simulink model "mcb_ipmsm_fwc_qep_f28379d"  (R2024b)
settings: Solver=FixedStepDiscrete  StartTime=0.0  StopTime=3  RelTol=1e-3  EnableMultiTasking=on
InitFcn:
  | mcb_ipmsm_fwc_qep_f28379d_data;
model workspace (MAT data in the model file):
  encoderResolution = 2000
  hallOffset = '0.5'
  indexOffset = 850
  polePairs = '4'
values from neighbouring files (symbols this model uses):
  dataType = 'single'    [mcb_e11_nonlin_fwc_data.m]    (also in mcb_e11_nonlin_setup.m; mcb_e11_params.m; mcb_ipmsm_fwc_qep_f28379d_data.m)
  inverter =     [e11_pmsmlut_full.mat]    (also in mcb_e11_nonlin_fwc_data.m = mcb_SetInverterParameters('BoostXL-DRV8305'); mcb_e11_nonlin_setup.m = S.inverter; mcb_ipmsm_fwc_qep_f28379d_data.m = mcb_SetInverterParameters('BoostXL-DRV8305'))
  lambda_pm = 0.0758825560532    [e11_pmsm_lut_data.mat]
  maxMotorCurrent = pmsm.I_rated    [mcb_e11_nonlin_fwc_data.m]    (also in mcb_e11_nonlin_setup.m; mcb_ipmsm_fwc_qep_f28379d_data.m)
  PI_params = mcb_SetControllerParameters(pmsm, inverter, PU_System, T_pwm, Ts, Ts_speed, Delays)    [mcb_e11_nonlin_fwc_data.m]    (also in mcb_e11_nonlin_setup.m; mcb_ipmsm_fwc_qep_f28379d_data.m = mcb_SetControllerParameters(pmsm,inverter,PU_System,T_pwm,Ts)
  pmsm = struct('I_rated', 433)    [e11_build_pmsmlut.m]    (also in e11_pmsmlut_full.mat = ; mcb_e11_nonlin_fwc_data.m = mcbPMSMUpdateLdLqFluxPM(pmsm, PMSMLUT, round(tmpmat(1,1)), r; mcb_e11_nonlin_setup.m = S.pmsm; mcb_ipmsm_fwc_qep_f28379d_data.m = mcb_SetPMSMMotorParameters('e11'))
  PU_System = mcb_SetPUSystem(pmsm, inverter)    [mcb_e11_nonlin_fwc_data.m]    (also in mcb_e11_nonlin_setup.m = struct(); mcb_ipmsm_fwc_qep_f28379d_data.m = mcb_SetPUSystem(pmsm,inverter))
  target = mcb_SetProcessorDetails('F28379D',PWM_frequency)    [mcb_ipmsm_fwc_qep_f28379d_data.m]
  Ts = T_pwm    (= 5e-05)    [mcb_e11_nonlin_fwc_data.m]    (also in mcb_e11_nonlin_setup.m; mcb_e11_params.m = ELEC.T_pwm; mcb_ipmsm_fwc_qep_f28379d_data.m)
  Ts_motor = T_pwm/2    (= 2.5e-05)    [mcb_e11_nonlin_fwc_data.m]    (also in mcb_e11_nonlin_setup.m; mcb_e11_params.m = ELEC.T_pwm/2; mcb_ipmsm_fwc_qep_f28379d_data.m)
  Ts_simulink = T_pwm/2    (= 2.5e-05)    [mcb_e11_nonlin_fwc_data.m]    (also in mcb_e11_nonlin_setup.m; mcb_e11_params.m = ELEC.T_pwm/2; mcb_ipmsm_fwc_qep_f28379d_data.m)
  Ts_speed = 30*Ts    (= 0.0015)    [mcb_e11_nonlin_fwc_data.m]    (also in mcb_e11_nonlin_setup.m; mcb_e11_params.m = 30*Ts; mcb_ipmsm_fwc_qep_f28379d_data.m)
undefined symbols (not defined in the file or in its folder): Down, GPTRIP1SEL, GPTRIP2SEL, TZ1, TZ2, Up
libraries: mcbcontrolslib x13, simulink x11, c280xlib x8, c2802xlib x7, slpidlib x4, mcbpositiondecoderlib x3, c2837xDlib x3, mcbpmsmnonlinearlib x2, svdschedulerlib x2, svdutilitieslib x1, mcbplantlib x1, autolibpmsminterior x1
(part 1 of 3)
settings Model: ExtModeTrigDuration=8  Creator=The MathWorks, Inc.  LastModifiedBy=The MathWorks, Inc.
settings SolverCC: AlgebraicLoopSolver=TrustRegion  MaxZcPerStep=1
settings DataIOCC: LimitDataPoints=on  SaveFormat=Array  SaveOutput=off  SaveTime=off  ReturnWorkspaceOutputs=off
settings OptimizationCC: DefaultUnderspecifiedDataType=single  OptimizeBlockIOStorage=off  BufferReuse=off  GlobalBufferReuse=off  ExpressionFolding=off  ExpressionDepthLimit=2147483647  LocalBlockOutputs=off  InitFltsAndDblsToZero=on  NoFixptDivByZeroProtection=on  EfficientFloat2IntCast=on  EfficientMapNaN2IntZero=off  LifeSpan=Inf  MaxStackSize=1024  OptimizeDataStoreBuffers=off  BusAssignmentInplaceUpdate=off  DenormalBehavior=FlushToZero  EfficientTunableParamExpr=on
settings DebuggingCC: ReadBeforeWriteMsg=DisableAll  WriteAfterWriteMsg=DisableAll  WriteAfterReadMsg=DisableAll  CheckSSInitialOutputMsg=off  SignalResolutionControl=TryResolveAllWithWarning  SolverPrmCheckMsg=warning  InheritedTsInSrcMsg=none  MultiTaskDSMMsg=none  MultiTaskCondExecSysMsg=none  TasksWithSamePriorityMsg=none  SigSpecEnsureSampleTimeMsg=none  IntegerOverflowMsg=none  ParameterPrecisionLossMsg=none  FcnCallInpInsideContextMsg=warning  UnconnectedInputMsg=warning  UnconnectedOutputMsg=warning  UnconnectedLineMsg=warning  AllowSymbolicDim=off  StateNameClashWarn=warning  SFUnexpectedBacktrackingDiag=warning  SFNoUnconditionalDefaultTransitionDiag=warning  SFExecutionAtInitializationDiag=none  IntegerSaturationMsg=none  ArithmeticOperatorsInVariantConditions=warning
settings HardwareCC: ProdBitPerChar=16  ProdBitPerInt=16  ProdBitPerPointer=32  ProdBitPerSizeT=32  ProdBitPerPtrDiffT=32  ProdLargestAtomicInteger=Integer  ProdLargestAtomicFloat=None  ProdWordSize=16  ProdLongLongMode=on  ProdHWDeviceType=Texas Instruments->C2000  TargetBitPerChar=16  TargetBitPerInt=16  TargetBitPerPointer=16  TargetLargestAtomicInteger=Integer  TargetIntDivRoundTo=Zero  TargetEndianess=LittleEndian  TargetWordSize=16  TargetHWDeviceType=TI C2000
settings ModelReferenceCC: EnableRefExpFcnMdlSchedulingChecks=on  PropagateSignalLabelsOutOfModel=off
settings SFSimCC: SimUseLocalCustomCode=off  MATLABDynamicMemAlloc=off  CustomCodeUndefinedFunction=UseInterfaceOnly
settings RTWCC: Description=Embedded Coder  SystemTargetFile=ert.tlc  HardwareBoard=TI Delfino F28379D LaunchPad  TemplateMakefile=ert_default_tmf  GenerateReport=on  RTWUseLocalCustomCode=off  Toolchain=Texas Instruments Code Composer Studio (C2000)  IncludeHyperlinkInReport=on  LaunchReport=on  GenerateTraceInfo=on  GenerateTraceReport=on  GenerateTraceReportSl=on  GenerateTraceReportSf=on  GenerateTraceReportEml=on  GPUComputeCapability=3.5  DLArmComputeVersion=19.05
settings CodeAppCC: IgnoreCustomStorageClasses=off  CustomSymbolStrType=$N$R$M  StateflowObjectComments=on  InternalIdentifier=Classic
settings ERTTargetCC: CodeReplacementLibrary=TI C28x  MultiwordLength=2048  ExtModeStaticAllocSize=10000  InlinedParameterPlacement=Hierarchical  ConvertIfToSwitch=off  SuppressUnreachableDefaultCases=off  MemSecPackage=tic2000demospkg
settings ConfigComp: CovMetricSettings=dw  CovSaveCumulativeToWorkspaceVar=on  CovSaveSingleToWorkspaceVar=on  CovExternalEMLEnable=off  CovSFcnEnable=off

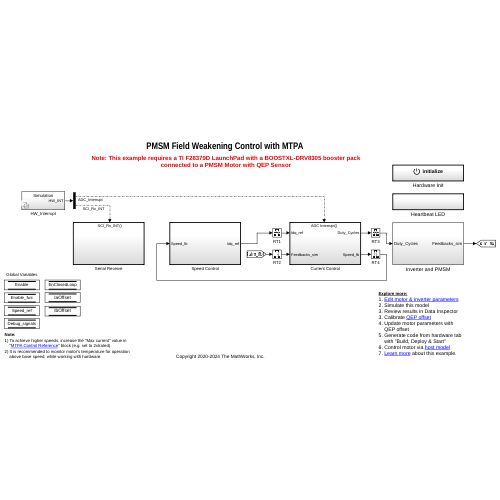
[thumbnail: Simulink's stored preview of the top-level diagram]
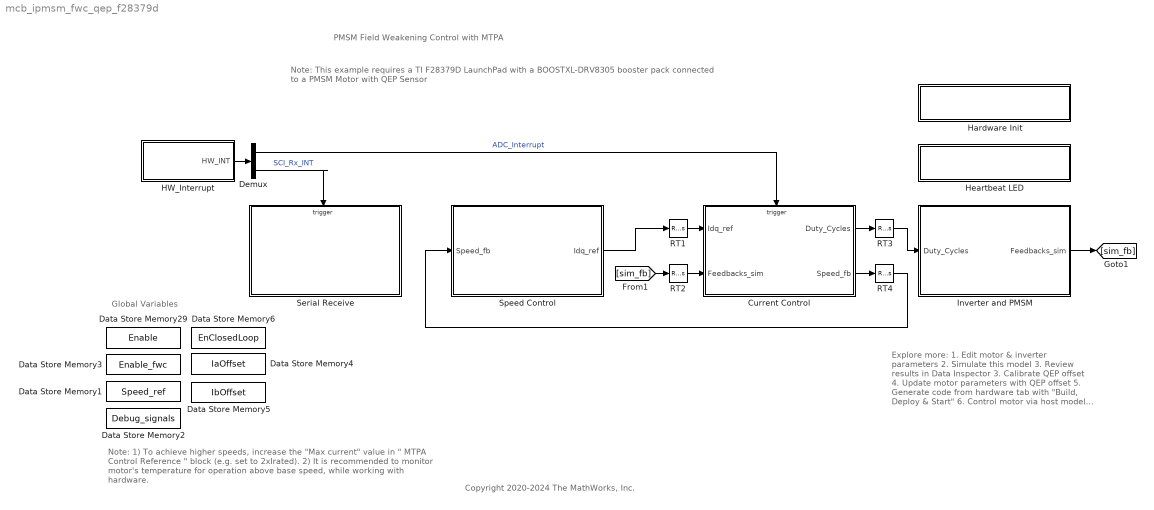
== system mcb_ipmsm_fwc_qep_f28379d ==
  note: Global Variables
  note: Copyright 2020-2024 The MathWorks, Inc.
  note: Explore more:
      | 1. Edit motor & inverter parameters
      | 2. Simulate this model
      | 3. Review results in Data Inspector
      | 3. Calibrate QEP offset
      | 4. Update motor parameters with
      | QEP offset
      | 5. Generate code from hardware tab
      | with "Build, Deploy & Start"
      | 6. Control motor via host model
      | 7. Learn more about this example.
  note: Note: This example requires a TI F28379D LaunchPad with a BOOSTXL-DRV8305 booster pack
      | connected to a PMSM Motor with QEP Sensor
  note: Note:
      | 1) To achieve higher speeds, increase the "Max current" value in
      | " MTPA Control Reference " block (e.g. set to 2xIrated).
      | 2) It is recommended to monitor motor's temperature for operation
      | above base speed, while working with hardware.
  note: PMSM Field Weakening Control with MTPA
  Current Control : Subsystem
      settings: RTWSystemCode=Nonreusable function
  Data Store Memory1 : DataStoreMemory  DataStoreName=Speed_ref  ReadBeforeWriteMsg=warning  WriteAfterWriteMsg=warning  WriteAfterReadMsg=warning  InitialValue=0.5  ShowAdditionalParam=off  OutDataTypeStr=dataType
  Data Store Memory2 : DataStoreMemory  DataStoreName=Debug_signals  ReadBeforeWriteMsg=warning  WriteAfterWriteMsg=warning  WriteAfterReadMsg=warning  InitialValue=5  ShowAdditionalParam=off  OutDataTypeStr=uint16
  Data Store Memory29 : DataStoreMemory  DataStoreName=Enable  ReadBeforeWriteMsg=warning  WriteAfterWriteMsg=warning  WriteAfterReadMsg=warning  ShowAdditionalParam=off  OutDataTypeStr=boolean
  Data Store Memory3 : DataStoreMemory  DataStoreName=Enable_fwc  ReadBeforeWriteMsg=warning  WriteAfterWriteMsg=warning  WriteAfterReadMsg=warning  ShowAdditionalParam=off  OutDataTypeStr=boolean
  Data Store Memory4 : DataStoreMemory  DataStoreName=IaOffset  InitialValue=inverter.CtSensAOffset  ShowAdditionalParam=off
  Data Store Memory5 : DataStoreMemory  DataStoreName=IbOffset  InitialValue=inverter.CtSensBOffset  ShowAdditionalParam=off
  Data Store Memory6 : DataStoreMemory  DataStoreName=EnClosedLoop  ReadBeforeWriteMsg=warning  WriteAfterWriteMsg=warning  WriteAfterReadMsg=warning  ShowAdditionalParam=off  OutDataTypeStr=boolean
  Demux : Demux  Outputs=2
  HW_Interrupt : Subsystem  Variant=on  VariantControlMode=sim codegen switching
  Hardware Init : Subsystem  TreatAsAtomicUnit=on
  Heartbeat LED : Subsystem  TreatAsAtomicUnit=on
  Inverter and PMSM : Subsystem
  RT1 : RateTransition  Deterministic=off
  RT2 : RateTransition  Deterministic=off
  RT3 : RateTransition  Deterministic=off
  RT4 : RateTransition  Deterministic=off  OutPortSampleTime=Ts_speed
  Serial Receive : Subsystem  SystemSampleTime=1e-3
  Speed Control : Subsystem  TreatAsAtomicUnit=on  SystemSampleTime=Ts_speed
      settings: RTWSystemCode=Nonreusable function
  wires:
  HW_Interrupt/1(HW_INT) -> Demux/1
  Demux/2 -> Serial Receive/Trigger  "SCI_Rx_INT"
  Demux/1 -> Current Control/Trigger  "ADC_Interrupt"
  Speed Control/1(Idq_ref) -> RT1/1
  [sim_fb] -> RT2/1
  Current Control/1(Duty_Cycles) -> RT3/1
  RT1/1 -> Current Control/1(Idq_ref)
  RT3/1 -> Inverter and PMSM/1(Duty_Cycles)
  Current Control/2(Speed_fb) -> RT4/1
  RT2/1 -> Current Control/2(Feedbacks_sim)
  Inverter and PMSM/1(Feedbacks_sim) -> [sim_fb]
  RT4/1 -> Speed Control/1(Speed_fb)

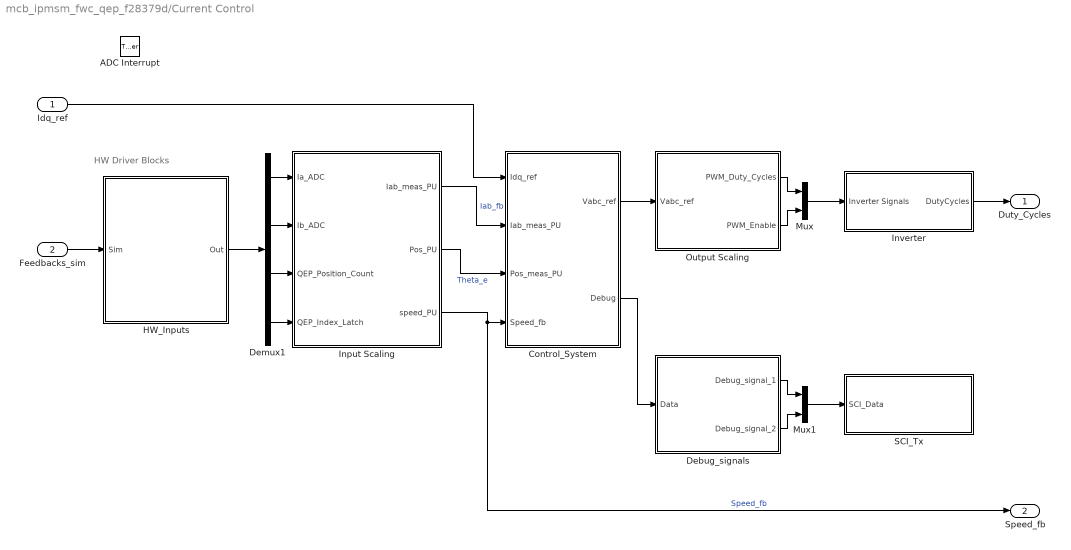
== system mcb_ipmsm_fwc_qep_f28379d/Current Control ==
  note: HW Driver Blocks
  Idq_ref : Inport
  Feedbacks_sim : Inport  Port=2
  ADC Interrupt : TriggerPort  TriggerType=function-call  VariantControl=Variant
  Control_System : Subsystem
  Debug_signals : Subsystem
  Demux1 : Demux
  HW_Inputs : Subsystem  Variant=on  VariantControlMode=sim codegen switching
  Input Scaling : Subsystem
  Inverter : Subsystem  Variant=on  VariantControlMode=sim codegen switching
  Mux : Mux  Inputs=2
  Mux1 : Mux  Inputs=2
  Output Scaling : Subsystem
  SCI_Tx : Subsystem  Variant=on  VariantControlMode=sim codegen switching
  Duty_Cycles : Outport  InitialOutput=0  VectorParamsAs1DForOutWhenUnconnected=off
  Speed_fb : Outport  Port=2  InitialOutput=0  VectorParamsAs1DForOutWhenUnconnected=off
  wires:
  Input Scaling/2(Pos_PU) -> Control_System/3(Pos_meas_PU)  "Theta_e"
  Input Scaling/3(speed_PU) -> Speed_fb/1, Control_System/4(Speed_fb)  "Speed_fb"
  Idq_ref/1 -> Control_System/1(Idq_ref)
  Control_System/1(Vabc_ref) -> Output Scaling/1(Vabc_ref)
  Input Scaling/1(Iab_meas_PU) -> Control_System/2(Iab_meas_PU)  "Iab_fb"
  Feedbacks_sim/1 -> HW_Inputs/1(Sim)
  Inverter/1(DutyCycles) -> Duty_Cycles/1
  Output Scaling/1(PWM_Duty_Cycles) -> Mux/1
  Output Scaling/2(PWM_Enable) -> Mux/2
  Mux/1 -> Inverter/1(Inverter Signals)
  HW_Inputs/1(Out) -> Demux1/1
  Demux1/2 -> Input Scaling/2(Ib_ADC)
  Demux1/1 -> Input Scaling/1(Ia_ADC)
  Demux1/3 -> Input Scaling/3(QEP_Position_Count)
  Demux1/4 -> Input Scaling/4(QEP_Index_Latch)
  Control_System/2(Debug) -> Debug_signals/1(Data)
  Mux1/1 -> SCI_Tx/1(SCI_Data)
  Debug_signals/1(Debug_signal_1) -> Mux1/1
  Debug_signals/2(Debug_signal_2) -> Mux1/2

== system mcb_ipmsm_fwc_qep_f28379d/HW_Interrupt ==
  Code generation : Subsystem  VariantControl=(codegen)
  Simulation : Subsystem  VariantControl=(sim)
  HW_INT : Outport  OutputFunctionCall=on

== system mcb_ipmsm_fwc_qep_f28379d/Hardware Init ==
  6PWM_Mode : Constant  Priority=1000  Value=0x3A16  OutDataTypeStr=uint16  SampleTime=-1
  ADC_Gain_Setting : Constant  Priority=1000  Value=inverter.SPI_Gain_Setting  OutDataTypeStr=uint16  SampleTime=-1
  Event Listener : EventListener  DisableCoverage=on  EventName=reset
  Mux : Mux  Inputs=2
  Variant Subsystem : Subsystem  Variant=on  VariantControlMode=sim codegen switching
  wires:
  6PWM_Mode/1 -> Mux/1
  ADC_Gain_Setting/1 -> Mux/2
  Mux/1 -> Variant Subsystem/1(In1)

== system mcb_ipmsm_fwc_qep_f28379d/Heartbeat LED ==
  note: Heartbeat LED 1HZ
  Heartbeat LED : Subsystem  Variant=on  VariantControlMode=sim codegen switching
  RED_LED : Constant  OutDataTypeStr=uint16  SampleTime=0.5
  wires:
  RED_LED/1 -> Heartbeat LED/1(In1)

== system mcb_ipmsm_fwc_qep_f28379d/Inverter and PMSM ==
  Duty_Cycles : Inport
  Codegeneration : Subsystem
  Simulation : Subsystem
  Variant Sink : VariantSink  VariantControlMode=sim codegen switching
  Variant Source : VariantSource  VariantControlMode=sim codegen switching
  Feedbacks_sim : Outport  VectorParamsAs1DForOutWhenUnconnected=off
  wires:
  Duty_Cycles/1 -> Variant Sink/1
  Variant Source/1 -> Feedbacks_sim/1
  Variant Sink/2 -> Simulation/1(Duty_Cycles)
  Simulation/1(Feedbacks) -> Variant Source/2
  Variant Sink/1 -> Codegeneration/1(Duty_Cycles)
  Codegeneration/1(Feedbacks) -> Variant Source/1

== system mcb_ipmsm_fwc_qep_f28379d/Serial Receive ==
  SCI_Rx_INT : TriggerPort  TriggerType=function-call  VariantControl=Variant
  Data Store Write : DataStoreWrite  DataStoreName=Enable  IndexOptions=Index vector (dialog)  Indices=1  OutputSizes=1
  Data Store Write1 : DataStoreWrite  DataStoreName=Debug_signals  IndexOptions=Index vector (dialog)  Indices=1  OutputSizes=1
  Data Store Write2 : DataStoreWrite  DataStoreName=Enable_fwc  IndexOptions=Index vector (dialog)  Indices=1  OutputSizes=1
  Data Store Write3 : DataStoreWrite  DataStoreName=Speed_ref  IndexOptions=Index vector (dialog)  Indices=1  OutputSizes=1
  Data_Conditioning_Rx : Subsystem  Variant=on
  SCI_Rx : Subsystem  Variant=on  VariantControlMode=sim codegen switching
  unParse : Subsystem
  wires:
  SCI_Rx/1(Out1) -> Data_Conditioning_Rx/1(In1)
  Data_Conditioning_Rx/1(Out1) -> Data Store Write3/1
  Data_Conditioning_Rx/2(Out2) -> unParse/1(Data)
  unParse/1(Enable_PWM) -> Data Store Write/1
  unParse/2(Enable_FWC) -> Data Store Write2/1
  unParse/3(Debug_signals) -> Data Store Write1/1

== system mcb_ipmsm_fwc_qep_f28379d/Speed Control ==
  Speed_fb : Inport
  Data Store Read : DataStoreRead  DataStoreName=Speed_ref  IndexOptions=Index vector (dialog)  Indices=1  OutputSizes=1
  Data Store Read1 : DataStoreRead  DataStoreName=Enable_fwc  IndexOptions=Index vector (dialog)  Indices=1  OutputSizes=1
  Id_ref : Constant  Value=0  OutDataTypeStr=Inherit: Inherit via back propagation  SampleTime=-1
  MTPA Control Reference : mcbcontrolslib/MTPA Control Reference  VariantSelect=Interior PMSM  polePairs=pmsm.p  Rs=pmsm.Rs  Ld=pmsm.Ld  Lq=pmsm.Lq  FluxPM=pmsm.FluxPM  ilimit=maxMotorCurrent  Vdc_input_select=Specify via dialog  V_dc=inverter.V_dc  Units=Per-Unit (PU)  N_base=pmsm.N_base  I_base=PU_System.I_base  T_base=0.74112  V_base=24/sqrt(3)  N_base_disp=4107  MTPAiterator=on  iterCount=10
  Mux1 : Mux  Inputs=2
  Mux2 : Mux  Inputs=2
  PI_Controller_Speed : Subsystem
  Saturation : Saturate  UpperLimit=pmsm.I_rated/PU_System.I_base  LowerLimit=-pmsm.I_rated/PU_System.I_base  RndMeth=Simplest
  StartUp_Logic : Subsystem
  Switch : Switch  Criteria=u2 > Threshold  SaturateOnIntegerOverflow=off  InputSameDT=off
  Idq_ref : Outport  VectorParamsAs1DForOutWhenUnconnected=off
  wires:
  MTPA Control Reference/2 -> Mux1/2
  PI_Controller_Speed/1(T_ref) -> MTPA Control Reference/1, Saturation/1
  Data Store Read/1 -> StartUp_Logic/1(Speed_Ref_In)  "speed_ref"
  Speed_fb/1 -> PI_Controller_Speed/2(Speed_fb)  "speed_fb"
  Mux1/1 -> Switch/1  "Idq_ref"
  StartUp_Logic/1(Speed_Ref_PU) -> MTPA Control Reference/2, PI_Controller_Speed/1(Speed_ref)
  MTPA Control Reference/1 -> Mux1/1
  Data Store Read1/1 -> Switch/2
  Mux2/1 -> Switch/3  "Idq_ref (No Field Weakening)"
  Id_ref/1 -> Mux2/1
  Switch/1 -> Idq_ref/1
  Saturation/1 -> Mux2/2

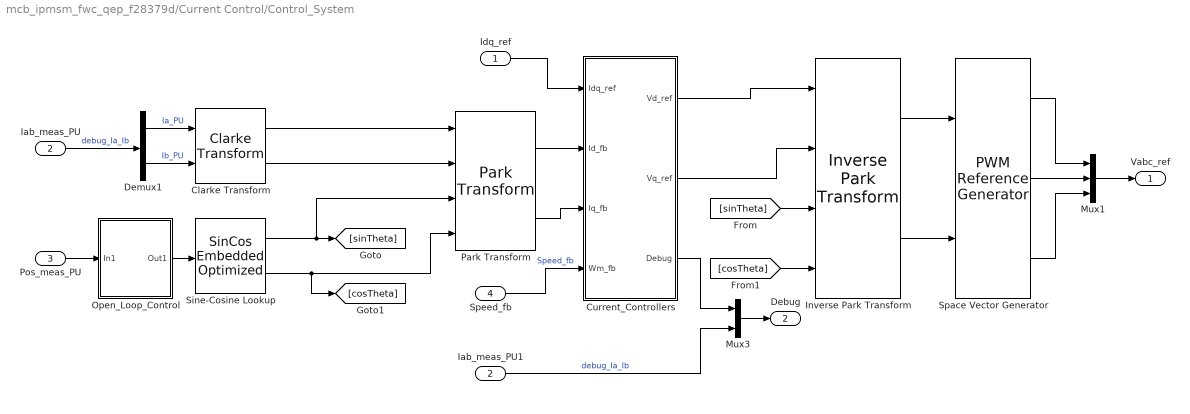
== system mcb_ipmsm_fwc_qep_f28379d/Current Control/Control_System ==
  Idq_ref : Inport
  Iab_meas_PU : Inport  Port=2
  Pos_meas_PU : Inport  Port=3
  Speed_fb : Inport  Port=4
  Clarke Transform : mcbcontrolslib/Clarke Transform  VariantControl=Variant2  PhaseInput=Two inputs  EnPowerInv=off
  Current_Controllers : Subsystem
  Demux1 : Demux  Outputs=2
  Iab_meas_PU1 : InportShadow  Port=2
  Inverse Park Transform : mcbcontrolslib/Inverse Park Transform  PhaseInput=Two inputs  AxisAlignment=D-axis  ThetaInput=Sine and Cosine electrical position  AngleInput=Per-unit  N_points=1024
  Mux1 : Mux  Inputs=3
  Mux3 : Mux  Inputs=2
  Open_Loop_Control : Subsystem
  Park Transform : mcbcontrolslib/Park Transform  PhaseInput=Two inputs  AxisAlignment=D-axis  ThetaInput=Sine and Cosine electrical position  AngleInput=Per-unit  N_points=1024
  Sine-Cosine Lookup : mcbcontrolslib/SinCos Embedded Optimized  LabelModeActiveChoice=MCB_Sin  OptforProc=off  ApproximationMethod=None  UserApproxMethod=Lookup  ApproxStatus=None  InterpMethod=Linear point-slope  NumberOfDataPoints=16  NumberOfIterations=11  RemoveProtectionAgainstOutOfRangeInput=off  TableDataTypeStr=Inherit: Inherit via input  AngleInput=Per-unit  ThetaDataType=single  N_points=1024  DatatypeInput=Inherit from input  Datatype=single
  Space Vector Generator : mcbcontrolslib/PWM Reference Generator  inSignal=Valphabeta  modType=SVM: space vector modulation
  Vabc_ref : Outport  VectorParamsAs1DForOutWhenUnconnected=off
  Debug : Outport  Port=2  VectorParamsAs1DForOutWhenUnconnected=off
  wires:
  Park Transform/1 -> Current_Controllers/2(Id_fb)
  Park Transform/2 -> Current_Controllers/3(Iq_fb)
  Inverse Park Transform/1 -> Space Vector Generator/1
  Inverse Park Transform/2 -> Space Vector Generator/2
  Sine-Cosine Lookup/1 -> Park Transform/3, [sinTheta]
  Sine-Cosine Lookup/2 -> Park Transform/4, [cosTheta]
  [cosTheta] -> Inverse Park Transform/4
  [sinTheta] -> Inverse Park Transform/3
  Clarke Transform/2 -> Park Transform/2
  Clarke Transform/1 -> Park Transform/1
  Idq_ref/1 -> Current_Controllers/1(Idq_ref)
  Space Vector Generator/1 -> Mux1/1
  Space Vector Generator/2 -> Mux1/2
  Current_Controllers/1(Vd_ref) -> Inverse Park Transform/1
  Current_Controllers/2(Vq_ref) -> Inverse Park Transform/2
  Pos_meas_PU/1 -> Open_Loop_Control/1(In1)
  Space Vector Generator/3 -> Mux1/3
  Mux1/1 -> Vabc_ref/1
  Demux1/1 -> Clarke Transform/1  "Ia_PU"
  Demux1/2 -> Clarke Transform/2  "Ib_PU"
  Iab_meas_PU/1 -> Demux1/1  "debug_Ia_Ib"
  Speed_fb/1 -> Current_Controllers/4(Wm_fb)  "Speed_fb"
  Iab_meas_PU1/1 -> Mux3/2  "debug_Ia_Ib"
  Current_Controllers/3(Debug) -> Mux3/1
  Mux3/1 -> Debug/1
  Open_Loop_Control/1(Out1) -> Sine-Cosine Lookup/1

== system mcb_ipmsm_fwc_qep_f28379d/Current Control/Debug_signals ==
  Data : Inport
  Data Store Read : DataStoreRead  DataStoreName=Debug_signals  IndexOptions=Index vector (dialog)  Indices=1  OutputSizes=1
  Demux : Demux  Outputs=2
  Ia_Ib : Constant  Value=[9 10]  OutDataTypeStr=uint16  SampleTime=-1
  Id_control : Constant  Value=[3 4]  OutDataTypeStr=uint16  SampleTime=-1
  Iq_control : Constant  Value=[5 6]  OutDataTypeStr=uint16  SampleTime=-1
  Multiport Switch : MultiPortSwitch  Inputs=5  DiagnosticForDefault=Warning  OutDataTypeStr=uint16  RndMeth=Simplest  SaturateOnIntegerOverflow=off  InputSameDT=off
  Selector : Selector  InputPortWidth=10  IndexOptions=Index vector (port)  Indices=[1 3]  OutputSizes=1
  Torque_and_Power : Constant  Value=[7 8]  OutDataTypeStr=uint16  SampleTime=-1
  speed_control : Constant  Value=[1 2]  OutDataTypeStr=uint16  SampleTime=-1
  Debug_signal_1 : Outport
  Debug_signal_2 : Outport  Port=2
  wires:
  Data/1 -> Selector/1
  Demux/2 -> Debug_signal_2/1
  speed_control/1 -> Multiport Switch/2
  Selector/1 -> Demux/1
  Demux/1 -> Debug_signal_1/1
  Id_control/1 -> Multiport Switch/3
  Iq_control/1 -> Multiport Switch/4
  Torque_and_Power/1 -> Multiport Switch/5
  Ia_Ib/1 -> Multiport Switch/6
  Multiport Switch/1 -> Selector/2
  Data Store Read/1 -> Multiport Switch/1

== system mcb_ipmsm_fwc_qep_f28379d/Current Control/HW_Inputs ==
  Sim : Inport
  Sensor Driver Blocks (codegen) : Subsystem  VariantControl=(codegen)
  Sensor Driver Blocks (sim) : Subsystem  VariantControl=(sim)
  Out : Outport

== system mcb_ipmsm_fwc_qep_f28379d/Current Control/Input Scaling ==
  note: Current Measurements
  note: Position & Speed Measurements
  note: QEP
  Ia_ADC : Inport
  Ib_ADC : Inport  Port=2
  QEP_Position_Count : Inport  Port=3
  QEP_Index_Latch : Inport  Port=4
  " Calculate Position and Speed" : Subsystem
  Calculate Phase Currents : Subsystem
  IndexOffset : Constant  Value=pmsm.PositionOffset  OutDataTypeStr=dataType  SampleTime=-1
  Terminator : Terminator
  Iab_meas_PU : Outport
  Pos_PU : Outport  Port=2
  speed_PU : Outport  Port=3
  wires:
  " Calculate Position and Speed"/2(speed) -> speed_PU/1
  Calculate Phase Currents/1(Iab_meas_PU) -> Iab_meas_PU/1  "Iab_fb_PU"
  QEP_Position_Count/1 -> " Calculate Position and Speed"/1(QEP_Position_Count)
  " Calculate Position and Speed"/1(Theta_e) -> Pos_PU/1
  Ia_ADC/1 -> Calculate Phase Currents/1(Ia_ADC)
  Ib_ADC/1 -> Calculate Phase Currents/2(Ib_ADC)
  QEP_Index_Latch/1 -> " Calculate Position and Speed"/2(QEP_Index_Latch)
  IndexOffset/1 -> " Calculate Position and Speed"/3(Offset)
  " Calculate Position and Speed"/3(IndexFound) -> Terminator/1

== system mcb_ipmsm_fwc_qep_f28379d/Current Control/Inverter ==
  Inverter Signals : Inport
  Code Generation : Subsystem  VariantControl=(codegen)
  Simulation : Subsystem  VariantControl=(sim)
  DutyCycles : Outport  VectorParamsAs1DForOutWhenUnconnected=off

== system mcb_ipmsm_fwc_qep_f28379d/Current Control/Output Scaling ==
  Vabc_ref : Inport
  Constant : Constant  Value=0.5  OutDataTypeStr=dataType  SampleTime=-1
  Data Type Conversion : DataTypeConversion  OutDataTypeStr=dataType  SaturateOnIntegerOverflow=off  RndMeth=Floor
  Enable : DataStoreRead  DataStoreName=Enable  IndexOptions=Index vector (dialog)  Indices=1  OutputSizes=1
  One_by_Two : Gain  Gain=0.5  RndMeth=Simplest  OutDataTypeStr=Inherit: Same as input
  Sum : Sum  Inputs=|++
  PWM_Duty_Cycles : Outport
  PWM_Enable : Outport  Port=2
  wires:
  Constant/1 -> Sum/2
  Vabc_ref/1 -> One_by_Two/1
  Sum/1 -> PWM_Duty_Cycles/1
  Enable/1 -> Data Type Conversion/1  "PWM_En"
  One_by_Two/1 -> Sum/1
  Data Type Conversion/1 -> PWM_Enable/1

== system mcb_ipmsm_fwc_qep_f28379d/Current Control/SCI_Tx ==
  SCI_Data : Inport
  Code Generation : Subsystem  VariantControl=(codegen)
  Simulation : Subsystem  VariantControl=(sim)

== system mcb_ipmsm_fwc_qep_f28379d/HW_Interrupt/Code generation ==
  HWI_ADCB1_INT : svdschedulerlib/Hardware Interrupt v2  ISRGroup=ADC - Analog to Digital Converter  ISRName=ADCA1_INT  ISRNumber=32  NumEventsToServe=1  EventsList={'on','EOC event','1';'off','Overflow event','2';'off','Custom event','3'}  SelectedEvents={'event1'}  TaskPriority=30  DisablePreemption=off  ClearInterruptFlagsAtEndOfEvent=on  InterruptDefinitionFile=$(TARGET_ROOT)/registry/interrupts/F2837xS_interrupts.xml  HardwareBoard=F2837x  EnableSimPort=off
      settings: LibrarySourceBlock=c2000lib/Scheduling/Hardware Interrupt
  HWI_SCIA_RX_INT : svdschedulerlib/Hardware Interrupt v2  ISRGroup=ADC - Analog to Digital Converter  ISRName=ADCA1_INT  ISRNumber=32  NumEventsToServe=1  EventsList={'on','EOC event','1';'off','Overflow event','2';'off','Custom event','3'}  SelectedEvents={'event1'}  TaskPriority=50  DisablePreemption=on  ClearInterruptFlagsAtEndOfEvent=on  InterruptDefinitionFile=$(TARGET_ROOT)/registry/interrupts/F2837xS_interrupts.xml  HardwareBoard=F2837x  EnableSimPort=off
      settings: LibrarySourceBlock=c2000lib/Scheduling/Hardware Interrupt
  Mux : Mux  Inputs=2
  HW_INT : Outport
  wires:
  HWI_ADCB1_INT/1 -> Mux/1
  Mux/1 -> HW_INT/1
  HWI_SCIA_RX_INT/1 -> Mux/2

== system mcb_ipmsm_fwc_qep_f28379d/HW_Interrupt/Simulation ==
  ADCINT1 : simulink/Ports & Subsystems/Function-Call Generator  sample_time=Ts  numberOfIterations=1  DisallowWideOutput=off
  Mux : Mux  Inputs=2
  SCI_Rx_INT : simulink/Ports & Subsystems/Function-Call Generator  sample_time=0.1  numberOfIterations=1  DisallowWideOutput=off
  HW_INT : Outport
  wires:
  SCI_Rx_INT/1 -> Mux/2
  ADCINT1/1 -> Mux/1
  Mux/1 -> HW_INT/1

== system mcb_ipmsm_fwc_qep_f28379d/Hardware Init/Variant Subsystem ==
  In1 : Inport
  Code Generation : Subsystem  VariantControl=(codegen)
  Simulation : Subsystem  VariantControl=(sim)

== system mcb_ipmsm_fwc_qep_f28379d/Heartbeat LED/Heartbeat LED ==
  In1 : Inport
  Code generation : Subsystem  VariantControl=(codegen)
  Simulation : Subsystem  VariantControl=(sim)

== system mcb_ipmsm_fwc_qep_f28379d/Inverter and PMSM/Codegeneration ==
  Duty_Cycles : Inport
  Ground : Ground
  Terminator : Terminator
  Feedbacks : Outport  VectorParamsAs1DForOutWhenUnconnected=off
  wires:
  Duty_Cycles/1 -> Terminator/1
  Ground/1 -> Feedbacks/1

== system mcb_ipmsm_fwc_qep_f28379d/Inverter and PMSM/Simulation ==
  Duty_Cycles : Inport
  Average Inverter : Subsystem
  Interior PMSM : autolibpmsminterior/Interior PMSM  port_config=Torque  sim_type=Discrete  Ts=Ts_motor  P=pmsm.p  Rs=pmsm.Rs + inverter.R_board  Ldq=[pmsm.Ld pmsm.Lq]  KConstText=Permanent flux linkage constant (lambda_pm):  lambda_pm=pmsm.FluxPM  Ke=159.9771  mechanical=[pmsm.J, pmsm.B,0]  idq0=[0 0]  theta_init=0  omega_init=0  KConst=pmsm.FluxPM  lambda_pm_calc=pmsm.FluxPM  Kt=0.07  RefBlkName='autolibpmsminterior/Interior PMSM'  aMode=5
      settings: LibrarySourceBlock=mcblib/Electrical Systems/Motors/Interior PMSM
  Load_Profile (Torque) : Subsystem
  RT1 : RateTransition  Deterministic=off  OutPortSampleTime=Ts_simulink
  RT3 : RateTransition  Deterministic=off  OutPortSampleTime=Ts_simulink
  Rate Transition : RateTransition  Deterministic=off  OutPortSampleTime=Ts_motor
  Rate Transition1 : RateTransition  Deterministic=off  OutPortSampleTime=Ts_motor
  Sensor_Measurements : Subsystem
  Terminator : Terminator
  Feedbacks : Outport  VectorParamsAs1DForOutWhenUnconnected=off
  wires:
  Sensor_Measurements/1(Sim_fb) -> Feedbacks/1
  Load_Profile (Torque)/1(Load_Trq) -> Rate Transition1/1
  Rate Transition1/1 -> Interior PMSM/1
  Interior PMSM/2 -> RT1/1  "Iabc"
  Duty_Cycles/1 -> Average Inverter/1(Duty_abc)
  Interior PMSM/3 -> Terminator/1
  Average Inverter/1(Vabc) -> Rate Transition/1
  Rate Transition/1 -> Interior PMSM/2
  RT3/1 -> Sensor_Measurements/1(Info)
  Interior PMSM/1 -> RT3/1
  RT1/1 -> Sensor_Measurements/2(PhaseCurr)

== system mcb_ipmsm_fwc_qep_f28379d/Serial Receive/Data_Conditioning_Rx ==
  In1 : Inport
  Data_Type_Fixed_Point : Subsystem  VariantControl=~isequal(dataType, 'single')
  Data_Type_Float : Subsystem  VariantControl=isequal(dataType, 'single')
  Out1 : Outport
  Out2 : Outport  Port=2

== system mcb_ipmsm_fwc_qep_f28379d/Serial Receive/SCI_Rx ==
  Code Generation : Subsystem  Variant=on  VariantControl=(codegen)
  Simulation : Subsystem  VariantControl=(sim)
  Out1 : Outport

== system mcb_ipmsm_fwc_qep_f28379d/Serial Receive/unParse ==
  Data : Inport
  Bitwise Operator : simulink/Logic and Bit Operations/Bitwise Operator  logicop=AND  UseBitMask=on  BitMask=hex2dec('0001')  BitMaskRealWorld=Stored Integer
  Bitwise Operator1 : simulink/Logic and Bit Operations/Bitwise Operator  logicop=AND  UseBitMask=on  BitMask=hex2dec('00F0')  BitMaskRealWorld=Stored Integer
  Bitwise Operator2 : simulink/Logic and Bit Operations/Bitwise Operator  logicop=AND  UseBitMask=on  BitMask=hex2dec('0002')  BitMaskRealWorld=Stored Integer
  Data Type Conversion3 : DataTypeConversion  OutDataTypeStr=boolean  RndMeth=Simplest  SaturateOnIntegerOverflow=off
  Data Type Conversion4 : DataTypeConversion  OutDataTypeStr=uint16  RndMeth=Simplest  SaturateOnIntegerOverflow=off
  Data Type Conversion5 : DataTypeConversion  OutDataTypeStr=boolean  RndMeth=Simplest  SaturateOnIntegerOverflow=off
  Shift Arithmetic : ArithShift  BitShiftNumber=1
  Shift Arithmetic1 : ArithShift  BitShiftNumber=4
  Enable_PWM : Outport
  Enable_FWC : Outport  Port=2
  Debug_signals : Outport  Port=3
  wires:
  Bitwise Operator2/1 -> Shift Arithmetic/1
  Bitwise Operator1/1 -> Shift Arithmetic1/1
  Data/1 -> Bitwise Operator/1, Bitwise Operator2/1, Bitwise Operator1/1
  Bitwise Operator/1 -> Data Type Conversion3/1
  Data Type Conversion4/1 -> Debug_signals/1
  Shift Arithmetic1/1 -> Data Type Conversion4/1
  Data Type Conversion3/1 -> Enable_PWM/1
  Shift Arithmetic/1 -> Data Type Conversion5/1
  Data Type Conversion5/1 -> Enable_FWC/1

== system mcb_ipmsm_fwc_qep_f28379d/Speed Control/PI_Controller_Speed ==
  Speed_ref : Inport
  Speed_fb : Inport  Port=2
  AND : Logic  IconShape=distinctive  AllPortsSameDT=off  OutDataTypeStr=boolean
  Data Store Read1 : DataStoreRead  DataStoreName=Enable  IndexOptions=Index vector (dialog)  Indices=1  OutputSizes=1
  Data Store Read3 : DataStoreRead  DataStoreName=EnClosedLoop  IndexOptions=Index vector (dialog)  Indices=1  OutputSizes=1
  Discrete PI Controller with anti-windup & reset : slpidlib/PID Controller  Controller=PI  Form=Parallel  TimeDomain=Discrete-time  UseExternalTs=off  SampleTime=-1  IntegratorMethod=Forward Euler  FilterMethod=Forward Euler  ControllerParametersSource=external  P=1  I=1  UseKiTs=on  D=0  UseExternalDerivativeSource=off  N=100  UseFilter=on  TunerSelectOption=Transfer Function Based (PID Tuner App)  InitialConditionSource=external  InitialConditionForIntegrator=0  InitialConditionForFilter=0  DifferentiatorICPrevScaledInput=0  ExternalReset=level  TrackingMode=off  Kt=1  LimitOutput=on  SatLimitsSource=internal  UpperSaturationLimit=1  LowerSaturationLimit=-1  LinearizeAsGain=on  AntiWindupMode=clamping  Kb=1  LimitIntegrator=off  UpperIntegratorSaturationLimit=inf  LowerIntegratorSaturationLimit=-inf  RndMeth=Simplest  POutMin=[]  POutMax=[]  IOutMin=[]  IOutMax=[]  DOutMin=[]  DOutMax=[]  NOutMin=[]  NOutMax=[]  SumOutMin=[]  SumOutMax=[]  SaturationOutDataTypeStr=Inherit: Inherit via back propagation  SaturationOutMin=[]  SaturationOutMax=[]  PParamMin=[]  PParamMax=[]  IParamMin=[]  IParamMax=[]  DParamMin=[]  DParamMax=[]  NParamMin=[]  NParamMax=[]  KbParamMin=[]  KbParamMax=[]  KtParamMin=[]  KtParamMax=[]  KbOutMin=[]  KbOutMax=[]  KtOutMin=[]  KtOutMax=[]  IntegratorOutMin=[]  IntegratorOutMax=[]  FilterOutMin=[]  FilterOutMax=[]  SumI1OutMin=[]  SumI1OutMax=[]  SumI2OutMin=[]  SumI2OutMax=[]  SumI3OutMin=[]  SumI3OutMax=[]  SumI4OutMin=[]  SumI4OutMax=[]  SumDOutMin=[]  SumDOutMax=[]  DifferentiatorOutMin=[]  DifferentiatorOutMax=[]  FilterDiffOutCoefMin=[]  FilterDiffOutCoefMax=[]  ReciprocalOutMin=[]  ReciprocalOutMax=[]  SumDenOutMin=[]  SumDenOutMax=[]  SumNumOutMin=[]  SumNumOutMax=[]  DivideOutMin=[]  DivideOutMax=[]  UdiffTsProdOutMin=[]  UdiffTsProdOutMax=[]  NTsProdOutMin=[]  NTsProdOutMax=[]  UintegralTsProdOutMin=[]  UintegralTsProdOutMax=[]  UngainTsProdOutMin=[]  UngainTsProdOutMax=[]  ClampingZeroOutDataTypeStr=Inherit: Inherit via back propagation  ClampingZeroOutMin=[]  ClampingZeroOutMax=[]  FilterDenConstantOutDataTypeStr=Inherit: Inherit via back propagation  FilterDenConstantOutMin=[]  FilterDenConstantOutMax=[]  PCopyOutDataTypeStr=Inherit: Inherit via back propagation  PCopyOutMin=[]  PCopyOutMax=[]  NCopyOutDataTypeStr=Inherit: Inherit via back propagation  NCopyOutMin=[]  NCopyOutMax=[]  IntegratorContinuousStateAttributes=''  IntegratorStateMustResolveToSignalObject=off  IntegratorRTWStateStorageClass=Auto  FilterContinuousStateAttributes=''  FilterStateMustResolveToSignalObject=off  FilterRTWStateStorageClass=Auto  ParallelPVariant=ExternalParameters  IdealPVariant=Disabled  IVariant=ExternalParameters  DVariant=Disabled  IntegratorVariant=Discrete  SatVariant=Enabled  AWVariant=DiscClampingParallel  PCopyVariant=Disabled  TRVariant=Disabled  FdbkBlocksVariant=Forward  IdealPFdbkVariant=Disabled  SatFdbkVariant=Disabled  DerivativeFilterVariant=Disabled  NVariant=Disabled  NCopyVariant=Disabled_SignalSpec  FilterICVariant=Disabled  IntegratorICVariant=ExternalICs  ExternalResetVariant=ExternalReset  TRSumVariant=Passthrough  SumFdbkVariant=Disabled  SumVariant=Sum_PI  TsampFilterVariant=InternalTs  TsampNgainVariant=Passthrough  TsampIntegralVariant=Disabled_SignalSpec  ExternalSaturationOutDataTypeStr=Inherit: Same as second input  DerivativeSourceVariant=Disabled  PreIntVariant=InternalPreInt
  Ki1 : Constant  Value=PI_params.Ki_speed*Ts_speed  OutDataTypeStr=dataType  SampleTime=-1
  Ki2 : Constant  Value=0  OutDataTypeStr=dataType  SampleTime=-1
  Kp1 : Constant  Value=PI_params.Kp_speed  OutDataTypeStr=dataType  SampleTime=-1
  Logical Operator : Logic  Operator=NOT  IconShape=distinctive  AllPortsSameDT=off  OutDataTypeStr=boolean
  Sum : Sum  Inputs=|+-
  T_ref : Outport  VectorParamsAs1DForOutWhenUnconnected=off
  wires:
  Discrete PI Controller with anti-windup & reset/1 -> T_ref/1
  Ki1/1 -> Discrete PI Controller with anti-windup & reset/3
  Kp1/1 -> Discrete PI Controller with anti-windup & reset/2
  Speed_fb/1 -> Sum/2
  Sum/1 -> Discrete PI Controller with anti-windup & reset/1
  Logical Operator/1 -> Discrete PI Controller with anti-windup & reset/4
  AND/1 -> Logical Operator/1
  Ki2/1 -> Discrete PI Controller with anti-windup & reset/5
  Speed_ref/1 -> Sum/1
  Data Store Read3/1 -> AND/2
  Data Store Read1/1 -> AND/1

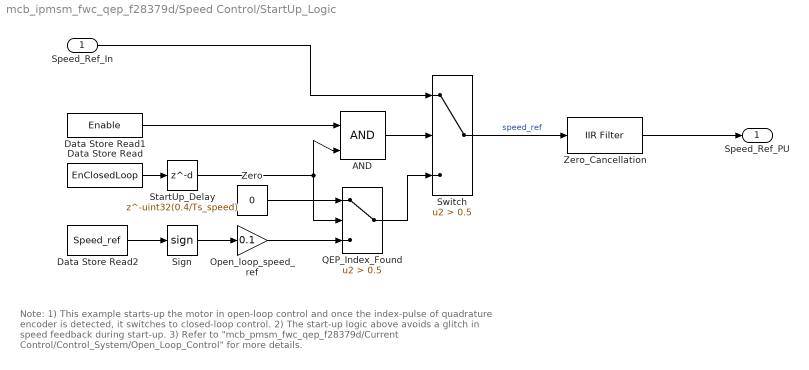
== system mcb_ipmsm_fwc_qep_f28379d/Speed Control/StartUp_Logic ==
  note: Note:
      | 1) This example starts-up the motor in open-loop control and once the index-pulse of quadrature encoder is detected, it switches to closed-loop control.
      | 2) The start-up logic above avoids a glitch in speed feedback during start-up.
      | 3) Refer to "mcb_pmsm_fwc_qep_f28379d/Current Control/Control_System/Open_Loop_Control" for more details.
  Speed_Ref_In : Inport
  AND : Logic  IconShape=distinctive  AllPortsSameDT=off  OutDataTypeStr=boolean
  Data Store Read : DataStoreRead  DataStoreName=EnClosedLoop  IndexOptions=Index vector (dialog)  Indices=1  OutputSizes=1
  Data Store Read2 : DataStoreRead  DataStoreName=Speed_ref  IndexOptions=Index vector (dialog)  Indices=1  OutputSizes=1
  Data Store Read1 : DataStoreRead  DataStoreName=Enable  IndexOptions=Index vector (dialog)  Indices=1  OutputSizes=1
  Open_loop_speed_ref : Gain  Gain=0.1  ParamDataTypeStr=dataType  OutDataTypeStr=dataType  RndMeth=Simplest
  QEP_Index_Found : Switch  Criteria=u2 > Threshold  Threshold=0.5  SaturateOnIntegerOverflow=off  InputSameDT=off
  Sign : Signum
  StartUp_Delay : Delay  DelayLength=uint32(0.4/Ts_speed)
  Switch : Switch  Criteria=u2 > Threshold  Threshold=0.5  SaturateOnIntegerOverflow=off  InputSameDT=off
  Zero : Constant  Value=0  OutDataTypeStr=dataType
  Zero_Cancellation : mcbcontrolslib/IIR Filter  VariantControl=Low Pass Filter  VariantSelect=Low-pass  FilterConstantInputType=Specify via dialog  Filter_constant=IIR_filter_speed.coeff_Ts_speed  advancedSettings=off  Ts=50e-6  cutOff_freq=1
  Speed_Ref_PU : Outport
  wires:
  Open_loop_speed_ref/1 -> QEP_Index_Found/3
  Speed_Ref_In/1 -> Switch/1
  AND/1 -> Switch/2
  Data Store Read1/1 -> AND/1
  Zero/1 -> QEP_Index_Found/1
  Data Store Read/1 -> StartUp_Delay/1
  Switch/1 -> Zero_Cancellation/1  "speed_ref"
  QEP_Index_Found/1 -> Switch/3
  StartUp_Delay/1 -> AND/2, QEP_Index_Found/2
  Sign/1 -> Open_loop_speed_ref/1
  Data Store Read2/1 -> Sign/1
  Zero_Cancellation/1 -> Speed_Ref_PU/1

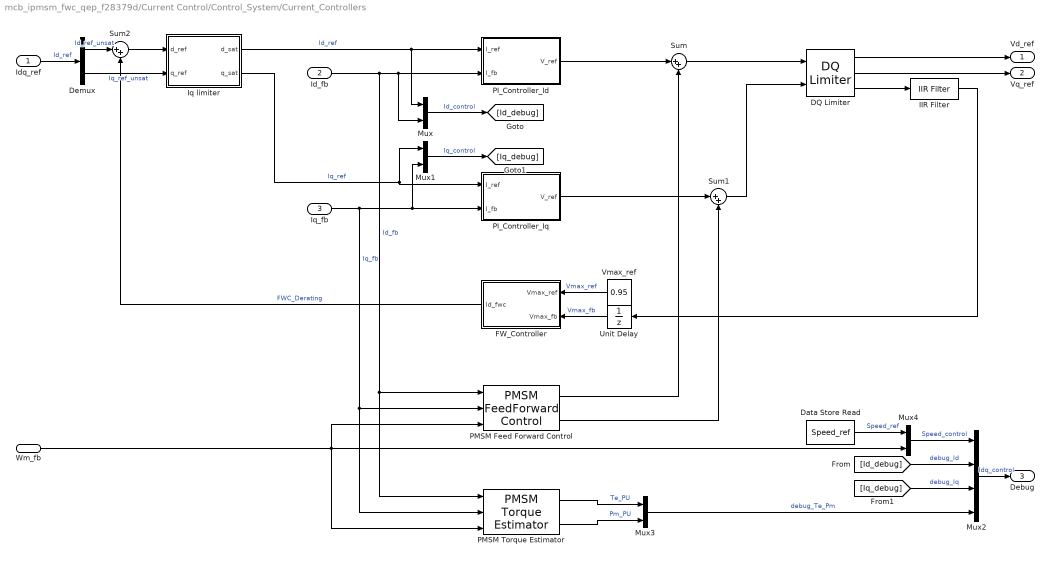
== system mcb_ipmsm_fwc_qep_f28379d/Current Control/Control_System/Current_Controllers ==
  Idq_ref : Inport
  Id_fb : Inport  Port=2
  Iq_fb : Inport  Port=3
  Wm_fb : Inport  Port=4
  DQ Limiter : mcbcontrolslib/DQ Limiter  satMethodInputType=Specify via dialog  satMethodSelected=D-Q equivalence  satLimitInputType=Specify via dialog  Vmax=0.95
  Data Store Read : DataStoreRead  DataStoreName=Speed_ref  IndexOptions=Index vector (dialog)  Indices=1  OutputSizes=1
  Demux : Demux  Outputs=2
  FW_Controller : Subsystem
  IIR Filter : mcbcontrolslib/IIR Filter  VariantControl=Low Pass Filter  VariantSelect=Low-pass  FilterConstantInputType=Specify via dialog  Filter_constant=0.01  advancedSettings=off  Ts=50e-6  cutOff_freq=32.1525
  Iq limiter : Subsystem
  Mux{,1,3..4} (4 alike) : Mux  Inputs=2
  Mux2 : Mux
  PI_Controller_Id : Subsystem
  PI_Controller_Iq : Subsystem
  PMSM Feed Forward Control : mcbpmsmnonlinearlib/PMSM FeedForward Control  polePairs=pmsm.p  nonLinearityChoice=Linear model with lumped parameters  Ld=pmsm.Ld  Lq=pmsm.Lq  FluxPM=pmsm.FluxPM  idVec=[-40, -20, 0, 20]  iqVec=[-40, -20, 0, 20, 40]  LdTable=0.2e-3 * ones(4, 5)  LqTable=0.2e-3 * ones(4, 5)  FluxPMTable=6.4e-3 * ones(4, 5)  FluxDTable=[-1.6,-1.6,-1.6,-1.6,-1.6;2.4,2.4,2.4,2.4,2.4;6.4,6.4,6.4,6.4,6.4;10.4,10.4,10.4,10.4,10.4]*1e-3  FluxQTable=[-8,-4,0,4,8;-8,-4,0,4,8;-8,-4,0,4,8;-8,-4,0,4,8]*1e-3  Vsat_input_select=Specify via dialog  v_sat=0.05*PU_System.V_base  Units=Per-Unit (PU)  V_base=PU_System.V_base  I_base=PU_System.I_base  N_base=PU_System.N_base  scaledTables=on
  PMSM Torque Estimator : mcbpmsmnonlinearlib/PMSM Torque Estimator  polePairs=pmsm.p  nonLinearityChoice=Linear model with lumped parameters  Ld=pmsm.Ld  Lq=pmsm.Lq  FluxPM=pmsm.FluxPM  idVec=[-40, -20, 0, 20]  iqVec=[-40, -20, 0, 20, 40]  LdTable=0.2e-3 * ones(4, 5)  LqTable=0.2e-3 * ones(4, 5)  FluxPMTable=6.4e-3 * ones(4, 5)  FluxDTable=[-1.6,-1.6,-1.6,-1.6,-1.6;2.4,2.4,2.4,2.4,2.4;6.4,6.4,6.4,6.4,6.4;10.4,10.4,10.4,10.4,10.4]*1e-3  FluxQTable=[-8,-4,0,4,8;-8,-4,0,4,8;-8,-4,0,4,8;-8,-4,0,4,8]*1e-3  Units=Per-Unit (PU)  V_base=PU_System.V_base  I_base=PU_System.I_base  N_base=PU_System.N_base  T_base=1.5  P_base=1.5  scaledTables=on
  Sum : Sum  Inputs=|++
  Sum1 : Sum  Inputs=|++
  Sum2 : Sum  Inputs=|++
  Unit Delay : UnitDelay  SampleTime=-1  HasFrameUpgradeWarning=on
  Vmax_ref : Constant  Value=0.95  OutDataTypeStr=dataType  SampleTime=-1
  Vd_ref : Outport  VectorParamsAs1DForOutWhenUnconnected=off
  Vq_ref : Outport  Port=2  VectorParamsAs1DForOutWhenUnconnected=off
  Debug : Outport  Port=3  VectorParamsAs1DForOutWhenUnconnected=off
  wires:
  Mux/1 -> [Id_debug]  "Id_control"
  Id_fb/1 -> PMSM Torque Estimator/1, PMSM Feed Forward Control/1, Mux/2, PI_Controller_Id/2(I_fb)  "Id_fb"
  Mux1/1 -> [Iq_debug]  "Iq_control"
  DQ Limiter/1 -> Vd_ref/1
  DQ Limiter/2 -> Vq_ref/1
  PI_Controller_Id/1(V_ref) -> Sum/1
  PMSM Torque Estimator/1 -> Mux3/1  "Te_PU"
  FW_Controller/1(Id_fwc) -> Sum2/2  "FWC_Derating"
  Vmax_ref/1 -> FW_Controller/1(Vmax_ref)  "Vmax_ref"
  Iq_fb/1 -> PMSM Torque Estimator/2, PMSM Feed Forward Control/2, PI_Controller_Iq/2(I_fb), Mux1/2  "Iq_fb"
  PI_Controller_Iq/1(V_ref) -> Sum1/1
  Sum1/1 -> DQ Limiter/2
  Sum/1 -> DQ Limiter/1
  Iq limiter/2(q_sat) -> PI_Controller_Iq/1(I_ref), Mux1/1  "Iq_ref"
  Unit Delay/1 -> FW_Controller/2(Vmax_fb)  "Vmax_fb"
  IIR Filter/1 -> Unit Delay/1
  DQ Limiter/3 -> IIR Filter/1
  PMSM Feed Forward Control/1 -> Sum/2
  PMSM Feed Forward Control/2 -> Sum1/2
  Idq_ref/1 -> Demux/1  "Id_ref"
  Mux2/1 -> Debug/1  "Idq_control"
  [Id_debug] -> Mux2/2  "debug_Id"
  [Iq_debug] -> Mux2/3  "debug_Iq"
  PMSM Torque Estimator/2 -> Mux3/2  "Pm_PU"
  Mux3/1 -> Mux2/4  "debug_Te_Pm"
  Mux4/1 -> Mux2/1  "Speed_control"
  Wm_fb/1 -> PMSM Torque Estimator/3, PMSM Feed Forward Control/3, Mux4/2
  Data Store Read/1 -> Mux4/1  "Speed_ref"
  Iq limiter/1(d_sat) -> PI_Controller_Id/1(I_ref), Mux/1  "Id_ref"
  Sum2/1 -> Iq limiter/1(d_ref)
  Demux/1 -> Sum2/1  "Id_ref_unsat"
  Demux/2 -> Iq limiter/2(q_ref)  "Iq_ref_unsat"

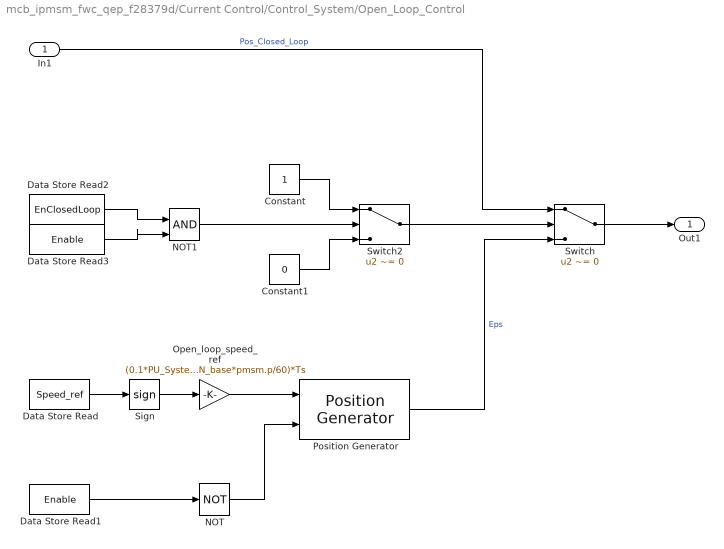
== system mcb_ipmsm_fwc_qep_f28379d/Current Control/Control_System/Open_Loop_Control ==
  In1 : Inport
  Constant : Constant  OutDataTypeStr=uint16
  Constant1 : Constant  Value=0  OutDataTypeStr=uint16
  Data Store Read : DataStoreRead  DataStoreName=Speed_ref  IndexOptions=Index vector (dialog)  Indices=1  OutputSizes=1
  Data Store Read1 : DataStoreRead  DataStoreName=Enable  IndexOptions=Index vector (dialog)  Indices=1  OutputSizes=1
  Data Store Read2 : DataStoreRead  DataStoreName=EnClosedLoop  IndexOptions=Index vector (dialog)  Indices=1  OutputSizes=1
  Data Store Read3 : DataStoreRead  DataStoreName=Enable  IndexOptions=Index vector (dialog)  Indices=1  OutputSizes=1
  NOT : Logic  Operator=NOT  IconShape=distinctive  AllPortsSameDT=off  OutDataTypeStr=boolean
  NOT1 : Logic  IconShape=distinctive  AllPortsSameDT=off  OutDataTypeStr=boolean
  Open_loop_speed_ref : Gain  Gain=(0.1*PU_System.N_base*pmsm.p/60)*Ts  ParamDataTypeStr=dataType  OutDataTypeStr=dataType  RndMeth=Simplest
  Position Generator : mcbcontrolslib/Position Generator  AngleOutput=Per-unit  ExternalReset=active high resets to zero  Offset=0
  Sign : Signum
  Switch : Switch  Criteria=u2 ~= 0  Threshold=0.1  SaturateOnIntegerOverflow=off  InputSameDT=off
  Switch2 : Switch  Criteria=u2 ~= 0  SaturateOnIntegerOverflow=off  InputSameDT=off
  Out1 : Outport
  wires:
  Constant1/1 -> Switch2/3
  Constant/1 -> Switch2/1
  In1/1 -> Switch/1  "Pos_Closed_Loop"
  Switch/1 -> Out1/1
  Open_loop_speed_ref/1 -> Position Generator/1
  Switch2/1 -> Switch/2
  Data Store Read/1 -> Sign/1
  Position Generator/1 -> Switch/3  "Eps"
  Data Store Read1/1 -> NOT/1
  NOT/1 -> Position Generator/2
  Data Store Read2/1 -> NOT1/1
  Data Store Read3/1 -> NOT1/2
  NOT1/1 -> Switch2/2
  Sign/1 -> Open_loop_speed_ref/1

== system mcb_ipmsm_fwc_qep_f28379d/Current Control/HW_Inputs/Sensor Driver Blocks (codegen) ==
  Sim : Inport
  ADC_B_IN2 : c2802xlib/ADC  blkParamProc=C2000_Type4  ADCModule=B  samplingMode=Single sample mode  ADCResolution=12-bit (Single-ended input)  useSOC1=SOC0  useSOC2=SOC0_SOC1  SOCAcquisitionWindow=15  SOCTriggerSource=ePWM1_ADCSOCA  SOCInterruptTrigger=No ADCINT  Ts=-1  dType=uint16  postInterrupt=on  interruptSel=ADCINT1  ADCINTContinuous=on  endma=off  chdma=1  conv1=ADCINA0  conv2=ADCINA0 and ADCINB0  conv1_Type4=ADCIN2  conv2_Type4=ADCIN0 and ADCIN1
  ADC_C_IN2 : c2802xlib/ADC  blkParamProc=C2000_Type4  ADCModule=C  samplingMode=Single sample mode  ADCResolution=12-bit (Single-ended input)  useSOC1=SOC0  useSOC2=SOC0_SOC1  SOCAcquisitionWindow=15  SOCTriggerSource=ePWM1_ADCSOCA  SOCInterruptTrigger=No ADCINT  Ts=-1  dType=uint16  postInterrupt=off  interruptSel=ADCINT1  ADCINTContinuous=on  endma=off  chdma=1  conv1=ADCINA0  conv2=ADCINA0 and ADCINB0  conv1_Type4=ADCIN2  conv2_Type4=ADCIN0 and ADCIN1
  Mux1 : Mux
  Optional_Read_SPI : Subsystem  Commented=on
  Terminator : Terminator
  eQEP : c280xlib/eQEP  useModule=eQEP1  pcInputmode=Quadrature-count  externalClockrate=2x resolution: Count the rising/falling edge  swapPolarityselection=Clockwise  qdfOutputport=off  qapPolarityselection=on  qbpPolarityselection=on  qipPolarityselection=on  qspPolarityselection=off  igatePolarityselection=off  sampleTime=-1  pcOutputport=on  pcMaximumvalue=2^16-1  indexInitializationcheck=off  indexInitializationevent=Rising edge  strobeInitializationcheck=off  strobeInitializationevent=Rising edge  softwareInitializationcheck=off  softwareInitializationsource=Set to init value at start up  softwareInitializationmode=on  pcInitialvalue=2147483648  pcResetmode=Reset on the first index event  ieloutputport=on  indexEventlatch=Falling edge  seloutputport=off  strobeEventlatch=Rising edge  pcefOutputport=off  enableEqepcapture=off  qctmrOutputport=off  qcprdOutputport=off  captureTimerprescaler=128  upEventprescaler=128  overflowErrorflag=off  directionErrorflag=off  captureTimerposition=On position counter read  unitTimerperiod=100000000  captureTimerlatch=off  capturePeriodlatch=off  positionCounterlatch=off  soenPolarityselection=off  spselPolarityselection=Index pin is used for sync output  compareValuesource=Specify via dialog  shadowMode=Load on QPOSCNT=0  compareValue=4294967295  syncOutputwidth=1  polaritySyncoutput=Active high  watchdogEnable=off  watchdogTimer=65535  outport1Datatype=auto  outport2Datatype=auto  outport3Datatype=auto  outport4Datatype=auto  outport5Datatype=auto  outport6Datatype=auto  outport7Datatype=auto  outport8Datatype=auto  outport9Datatype=auto  outport10Datatype=auto  outport11Datatype=auto  outport12Datatype=auto  eqepinterrupt_pce=off  eqepinterrupt_qpe=off  eqepinterrupt_qdc=off  eqepinterrupt_wto=off  eqepinterrupt_pcu=off  eqepinterrupt_pco=off  eqepinterrupt_pcr=off  eqepinterrupt_pcm=off  eqepinterrupt_sel=off  eqepinterrupt_iel=off  eqepinterrupt_uto=off  pheOutputport=off  watchdogOutputport=off  outport13Datatype=auto  outport14Datatype=auto
  Out : Outport
  wires:
  ADC_C_IN2/1 -> Mux1/1
  Mux1/1 -> Out/1
  ADC_B_IN2/1 -> Mux1/2
  Sim/1 -> Terminator/1
  eQEP/1 -> Mux1/3
  eQEP/2 -> Mux1/4

== system mcb_ipmsm_fwc_qep_f28379d/Current Control/HW_Inputs/Sensor Driver Blocks (sim) ==
  Sim : Inport
  Out : Outport
  wires:
  Sim/1 -> Out/1

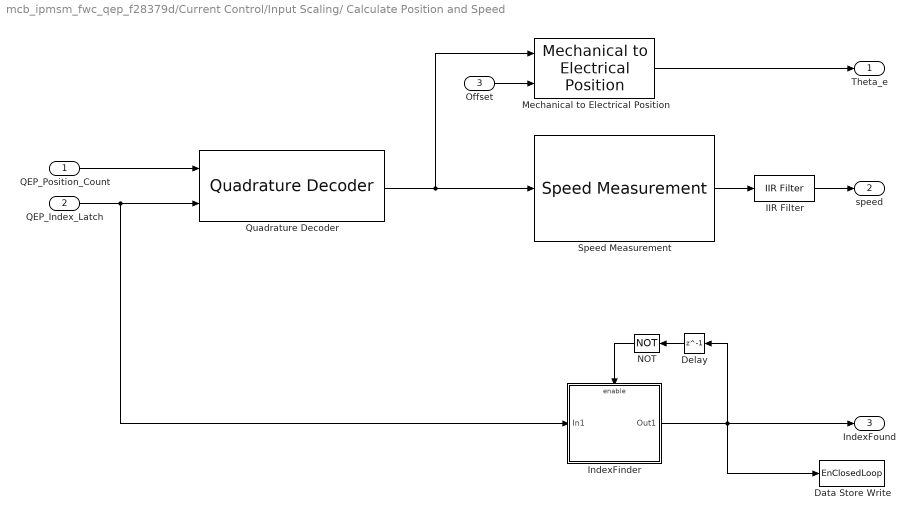
== system mcb_ipmsm_fwc_qep_f28379d/Current Control/Input Scaling/ Calculate Position and Speed ==
  QEP_Position_Count : Inport
  QEP_Index_Latch : Inport  Port=2
  Offset : Inport  Port=3
  Data Store Write : DataStoreWrite  DataStoreName=EnClosedLoop  IndexOptions=Index vector (dialog)  Indices=1  OutputSizes=1
  Delay : Delay  DelayLength=1
  IIR Filter : mcbcontrolslib/IIR Filter  VariantControl=Low Pass Filter  VariantSelect=Low-pass  FilterConstantInputType=Specify via dialog  Filter_constant=IIR_filter_speed.coeff_Ts  advancedSettings=off  Ts=50e-6  cutOff_freq=1
  IndexFinder : Subsystem
  Mechanical to Electrical Position : mcbpositiondecoderlib/Mechanical to Electrical Position  PolePairsInputType=Specify via dialog  NrPP=pmsm.p  selectedRange=Per unit  MechOfstInputType=Input port  mechOffsetIn=0  maxAngleIn=1  InputDataType=dataType  VariantSelect=floating-point
  NOT : Logic  Operator=NOT  AllPortsSameDT=off  OutDataTypeStr=boolean
  Quadrature Decoder : mcbpositiondecoderlib/Quadrature Decoder  EncoderSlitsPerRevolution=pmsm.QEPSlits  EncoderCountsPerSlit=4  CounterSize=16 bits  ExternalIndexCount=on  PositionUnit=Per unit  PositionDataType=dataType  ParameterInputType=off  CountsPerRevInverseDataType=single
  Speed Measurement : mcbpositiondecoderlib/Speed Measurement  PositionUnit=Per unit  PositionScalingDatatype=uint32  SpeedCalculationMode=Time interval for speed calculation  SampleTimeAsync=Ts  MaximumApplicationSpeed=6000  SpeedResolution=5e-6  DelayLength=20  MaximumMeasurableSpeed=-0.98352  MeasurableSpeedResolution=7.6757e-12  SpeedUnit=Per unit based on dialog  PerUnitSpeed=PU_System.N_base  SpeedDataType=dataType
  Theta_e : Outport  VectorParamsAs1DForOutWhenUnconnected=off
  speed : Outport  Port=2  VectorParamsAs1DForOutWhenUnconnected=off
  IndexFound : Outport  Port=3  InitialOutput=0  VectorParamsAs1DForOutWhenUnconnected=off
  wires:
  Speed Measurement/1 -> IIR Filter/1
  Mechanical to Electrical Position/1 -> Theta_e/1
  QEP_Position_Count/1 -> Quadrature Decoder/1
  Quadrature Decoder/1 -> Mechanical to Electrical Position/1, Speed Measurement/1
  Offset/1 -> Mechanical to Electrical Position/2
  IIR Filter/1 -> speed/1
  Delay/1 -> NOT/1
  NOT/1 -> IndexFinder/Enable
  QEP_Index_Latch/1 -> IndexFinder/1(In1), Quadrature Decoder/2
  IndexFinder/1(Out1) -> Data Store Write/1, Delay/1, IndexFound/1

== system mcb_ipmsm_fwc_qep_f28379d/Current Control/Input Scaling/Calculate Phase Currents ==
  Ia_ADC : Inport
  Ib_ADC : Inport  Port=2
  Add : Sum  Inputs=-+
  Data Store Read1 : DataStoreRead  DataStoreName=IaOffset  IndexOptions=Index vector (dialog)  Indices=1  OutputSizes=1
  Data Store Read2 : DataStoreRead  DataStoreName=IbOffset  IndexOptions=Index vector (dialog)  Indices=1  OutputSizes=1
  Data Type Conversion : DataTypeConversion  OutDataTypeStr=int32  ConvertRealWorld=Stored Integer (SI)  RndMeth=Simplest  SaturateOnIntegerOverflow=off
  Data_Type : Subsystem  Variant=on
  Inverting / Non-inverting Current measurement amplifieer : Gain  Gain=inverter.invertingAmp  RndMeth=Simplest  OutDataTypeStr=Inherit: Same as input
  Mux : Mux  Inputs=2
  Mux1 : Mux  Inputs=2
  Iab_meas_PU : Outport  VectorParamsAs1DForOutWhenUnconnected=off
  wires:
  Data Type Conversion/1 -> Add/2
  Add/1 -> Data_Type/1(In1)
  Ia_ADC/1 -> Mux/1
  Ib_ADC/1 -> Mux/2
  Mux/1 -> Data Type Conversion/1
  Mux1/1 -> Add/1
  Data Store Read1/1 -> Mux1/1
  Data Store Read2/1 -> Mux1/2
  Data_Type/1(Out1) -> Inverting / Non-inverting Current measurement amplifieer/1
  Inverting / Non-inverting Current measurement amplifieer/1 -> Iab_meas_PU/1
